simulink model "active_f2800137"  (R2024b)
settings: Solver=FixedStepDiscrete  StartTime=0.0  StopTime=inf  FixedStep=100e-6  RelTol=1e-3
model workspace (MAT data in the model file):
  ADC_FS = 4096
  ADC_VREF = 3.3
  G_CONST = 200
  IL_RATIO = 0.59
  IL_ZERO_V = 2.6365
  IPV_RATIO = 0.594
  IPV_ZERO_V = 2.6202
  ISENS_VPA = 0.1
  VOUT_RATIO = 0.021
  VPV_RATIO = 0.059
undefined symbols (not defined in the file or in its folder): Down, GPTRIP1SEL, GPTRIP2SEL, TZ1, TZ2, Up
libraries: c2802xlib x6, c2000lib x1, simulink x1
settings Model: ExtModeTrigDuration=8  Creator=YOGA Slim 7 Pro  LastModifiedBy=YOGA Slim 7 Pro
settings DataIOCC: SaveOutput=off  SignalLogging=off  DSMLogging=off  SaveTime=off  ReturnWorkspaceOutputs=off
settings OptimizationCC: DefaultParameterBehavior=Inlined  DefaultUnderspecifiedDataType=single  EnhancedBackFolding=on  PassReuseOutputArgsAs=Individual arguments  MaxStackSize=1024  OptimizeBlockOrder=speed  DifferentSizesBufferReuse=on  OptimizationCustomize=off  EfficientTunableParamExpr=on
settings DebuggingCC: ParameterTunabilityLossMsg=error
settings HardwareCC: ProdBitPerChar=16  ProdBitPerInt=16  ProdBitPerPointer=32  ProdBitPerSizeT=32  ProdBitPerPtrDiffT=32  ProdLargestAtomicInteger=Integer  ProdLargestAtomicFloat=None  ProdWordSize=16  ProdLongLongMode=on  ProdHWDeviceType=Texas Instruments->C2000
settings SFSimCC: MATLABDynamicMemAlloc=off
settings RTWCC: Description=Embedded Coder  SystemTargetFile=ert.tlc  HardwareBoard=TI F2800137 LaunchPad  TemplateMakefile=ert_default_tmf  Toolchain=Texas Instruments Code Composer Studio (C2000)  CodeProfilingSaveOptions=MetricsOnly
settings CodeAppCC: ForceParamTrailComments=on  IgnoreCustomStorageClasses=off  OperatorAnnotations=on  SimulinkDataObjDesc=on  SFDataObjDesc=on  InsertBlockDesc=on
settings ERTTargetCC: CodeReplacementLibrary=TI C28x  ExtModeTransport=4  ExtModeStaticAlloc=on  ExtModeAutomaticAllocSize=off  ExtModeStaticAllocSize=1000  ExtModeMexFile=ext_xcp  ExtModeIntrfLevel=Level2 - Open

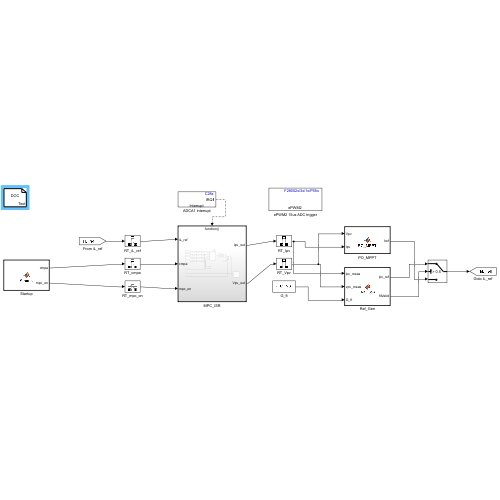
[thumbnail: Simulink's stored preview of the top-level diagram]
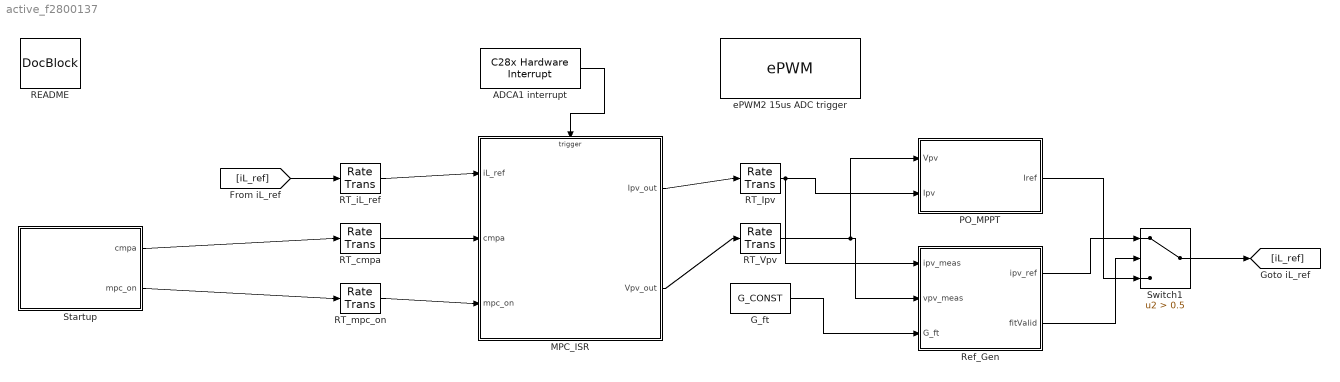
== system active_f2800137 ==
  ADCA1 interrupt : c2000lib/Scheduling/C28x Hardware Interrupt  irqnumbers=1  pienumbers=1  irqpriorities=30  irqpreempts=0  showinput=off  dspchiptype=C280X
  G_ft : Constant  Value=G_CONST  OutDataTypeStr=single  SampleTime=100e-6
  MPC_ISR : Subsystem  TreatAsAtomicUnit=on
  PO_MPPT : MATLAB Function  TreatAsAtomicUnit=on
  README : simulink/Model-Wide Utilities/DocBlock  DocumentType=Text
      content=|
      | active_f2800137 - controller of active.slx for the TMS320F2800137
      |
      | Gate output : ePWM1A = GPIO0
      | ADC-A inputs: iL=ADCIN2  Vin(Vpv)=ADCIN6  Vout=ADCIN3  Ipv=ADCIN5
      | Irradiance  : constant G_CONST = 200 W/m^2 (model workspace)
      | Scaling     : Model Explorer > Model Workspace
      |
      | MPC_Boost runs every 15 us in the ADCA1 interrupt (ePWM2 starts the
      | conversions). PO_MPPT and Ref_Gen run every 100 us. For t < 0.06 s
      | ePWM1A outputs the 30 kHz start-up PWM; afterwards the MPC switching
      | state S drives the pin directly.
  RT_Ipv : RateTransition  Deterministic=off  OutPortSampleTime=100e-6
  RT_Vpv : RateTransition  Deterministic=off  OutPortSampleTime=100e-6
  RT_cmpa : RateTransition  Deterministic=off  InitialCondition=200  OutPortSampleTimeOpt=Inherit
  RT_iL_ref : RateTransition  Deterministic=off  InitialCondition=4.9  OutPortSampleTimeOpt=Inherit
  RT_mpc_on : RateTransition  Deterministic=off  OutPortSampleTimeOpt=Inherit
  Ref_Gen : MATLAB Function  TreatAsAtomicUnit=on
  Startup : MATLAB Function  TreatAsAtomicUnit=on
  Switch1 : Switch  Criteria=u2 > Threshold  Threshold=0.5  SaturateOnIntegerOverflow=off  InputSameDT=off
  ePWM2 15us ADC trigger : c2802xlib/ePWM  PwmType=C2000_Type4_F28002x  useModule=ePWM2  ePWMxLINKTBPRD=Not Linked  periodUnits=Clock cycles  timerSource=Specify via dialog  timerPeriod_clk=1799  timerPeriod_sec=0.0001  tbshadow=Counter equals to zero  countingMode=Up  phaseActiveEnable=Disable  phaseDirection=Count down after sync  phaseActive=0  synchronizationEnable=off  dcaevt1Sync=off  dcbevt1Sync=off  synchronizationOption=Disable  dcbevt1SyncOut=off  dcaevt1SyncOut=off  cmpdSyncOut=off  cmpcSyncOut=off  cmpbSyncOut=off  zeroSyncOut=off  swfSyncOut=off  perSynchronizationOption=Counter equals to period (CTR=PRD)  clockPrescale=1  HSclockPrescale=1  enswap=off  ePWMxAStatus=off  ePWMxAactionLogic1=Set  ePWMxAactionLogic2=Clear  ePWMxAactionLogic3=Clear  ePWMxAactionLogic4=Set  ePWMxAactionLogic5=Do nothing  ePWMxAactionLogic6=Do nothing  ePWMxACSFenable=off  ePWMxACSFvalue=Forcing disable  ePWMxASFreload=Zero  ePWMxBStatus=off  ePWMxBactionLogic1=Set  ePWMxBactionLogic2=Clear  ePWMxBactionLogic3=Do nothing  ePWMxBactionLogic4=Do nothing  ePWMxBactionLogic5=Clear  ePWMxBactionLogic6=Set  ePWMxBCSFenable=off  ePWMxBCSFvalue=Forcing disable  ePWMxBSFreload=Zero  ePWNxBOutWay=off  ePWMxLINKCMPA=Not Linked  CMPAUnits=Clock cycles  CMPASource=Specify via dialog  CMPAValue_per=50  CMPAValue_clk=32000  enCMPAshadow=Counter equals to zero (CTR=Zero)  ePWMxLINKCMPB=Not Linked  CMPBUnits=Clock cycles  CMPBSource=Specify via dialog  CMPBValue_per=50  CMPBValue_clk=32000  enCMPBshadow=Counter equals to zero (CTR=Zero)  ePWMxLINKCMPC=Not Linked  CMPCUnits=Clock cycles  CMPCSource=Specify via dialog  CMPCValue_per=50  CMPCValue_clk=32000  enCMPCshadow=Counter equals to zero (CTR=Zero)  ePWMxLINKCMPD=Not Linked  CMPDUnits=Clock cycles  CMPDSource=Specify via dialog  CMPDValue_per=50  CMPDValue_clk=32000  enCMPDshadow=Counter equals to zero (CTR=Zero)  enableDBePWMxA=off  enableDBePWMxB=off  enhalfcycle=off  DBpolarity=Active high (AH)  DBedgeDelay=Positive  DBSource_ePWMxA=ePWMxA  DBSource_ePWMxB=ePWMxA  DBPeriodUnits=Clock cycles  DBperiodSource=Specify via dialog  REDperiod=0  FEDperiod=0  REDperiod_sec=0  FEDperiod_sec=0  LoadModeDBRED=Immediate without using shadow  LoadModeDBFED=Immediate without using shadow  adcstartModuleA=on  adcrequestEventA=First event  adcstartEventA=Counter equals to zero (CTR=Zero)  adcstartEventA_type2=Counter equals to zero (CTR=Zero)  adcstartModuleB=off  adcrequestEventB=First event  adcstartEventB=Counter equals to zero (CTR=Zero)  adcstartEventB_type2=Counter equals to zero (CTR=Zero)  intEn=off  intPrd=First event  intSel=Counter equals to zero (CTR=Zero)  intSel_type2=Counter equals to zero (CTR=Zero)  hrpe=off  enHRPWM=off  HRPWM_LoadMode=Counter equals to period (CTR=PRD)  HRPWM_CTLMode=Duty or Period control mode  HRPWM_EDGMode=Both edge  hrpeb=off  enHRPWMB=off  HRPWM_LoadModeB=Counter equals to zero (CTR=ZERO)  HRPWM_CTLModeB=Duty or Period control mode  HRPWM_EDGModeB=Both edge  enHRDBRED=off  enHRDBFED=off  enSFO=on  enautoconv=on  chopperEnable=off  chopperFrequency=1  chopperFirstwidth=1  chopperDuty=12.5%  tripZonesource=Specify via dialog  tzselOSHT1=off  tzselOSHT2=off  tzselOSHT3=off  tzselOSHT4=off  tzselOSHT5=off  tzselOSHT6=off  tzselOSHDCAEV1=off  tzselOSHDCBEV1=off  tzselCBC1=off  tzselCBC2=off  tzselCBC3=off  tzselCBC4=off  tzselCBC5=off  tzselCBC6=off  tzselCBCDCAEV2=off  tzselCBCDCBEV2=off  enTzOstIntr=off  enTzCbcIntr=off  enTzDCAEVT1Intr=off  enTzDCAEVT2Intr=off  enTzDCBEVT1Intr=off  enTzDCBEVT2Intr=off  tzclrCBCLatch=Counter equals to zero (CTR=Zero)  ePWMxAforced=No action  ePWMxBforced=No action  DCAEVT1forced=High  DCBEVT1forced=High  DCAEVT2forced=Low  DCBEVT2forced=Low  dcah=Trip Zone 1 input (TZ1)  dcal=Trip Zone 1 input (TZ1)  dcbh=Trip Zone 1 input (TZ1)  dcbl=Trip Zone 1 input (TZ1)  dcah_type2=GPTRIP1SEL/(TZ1)  dcal_type2=GPTRIP2SEL/(TZ2)  dcbh_type2=GPTRIP1SEL/(TZ1)  dcbl_type2=GPTRIP2SEL/(TZ2)  gendcaevt1=Event disabled  gendcaevt2=Event disabled  gendcbevt1=Event disabled  gendcbevt2=Event disabled  dcaevt1src=DCAEVT1 with sync  dcaevt2src=DCAEVT2 with sync  dcbevt1src=DCBEVT1 with sync  dcbevt2src=DCBEVT2 with sync  pulsesel=Counter equals to zero (CTR=Zero)  blankinv=off  blankoffset=0  blankwidth=0  evsrcsel=Filtered version of DCAEVT1 (DCAEVT1FILT)  encape=off
      settings: LibrarySourceBlock=c280013xlib/ePWM
  wires:
  ADCA1 interrupt/1 -> MPC_ISR/Trigger
  Startup/1(cmpa) -> RT_cmpa/1
  Startup/2(mpc_on) -> RT_mpc_on/1
  RT_iL_ref/1 -> MPC_ISR/1(iL_ref)
  RT_cmpa/1 -> MPC_ISR/2(cmpa)
  RT_mpc_on/1 -> MPC_ISR/3(mpc_on)
  MPC_ISR/1(Ipv_out) -> RT_Ipv/1
  MPC_ISR/2(Vpv_out) -> RT_Vpv/1
  RT_Vpv/1 -> PO_MPPT/1(Vpv), Ref_Gen/2(vpv_meas)
  RT_Ipv/1 -> PO_MPPT/2(Ipv), Ref_Gen/1(ipv_meas)
  G_ft/1 -> Ref_Gen/3(G_ft)
  Ref_Gen/1(ipv_ref) -> Switch1/1
  Ref_Gen/2(fitValid) -> Switch1/2
  PO_MPPT/1(Iref) -> Switch1/3
  Switch1/1 -> [iL_ref]
  [iL_ref] -> RT_iL_ref/1

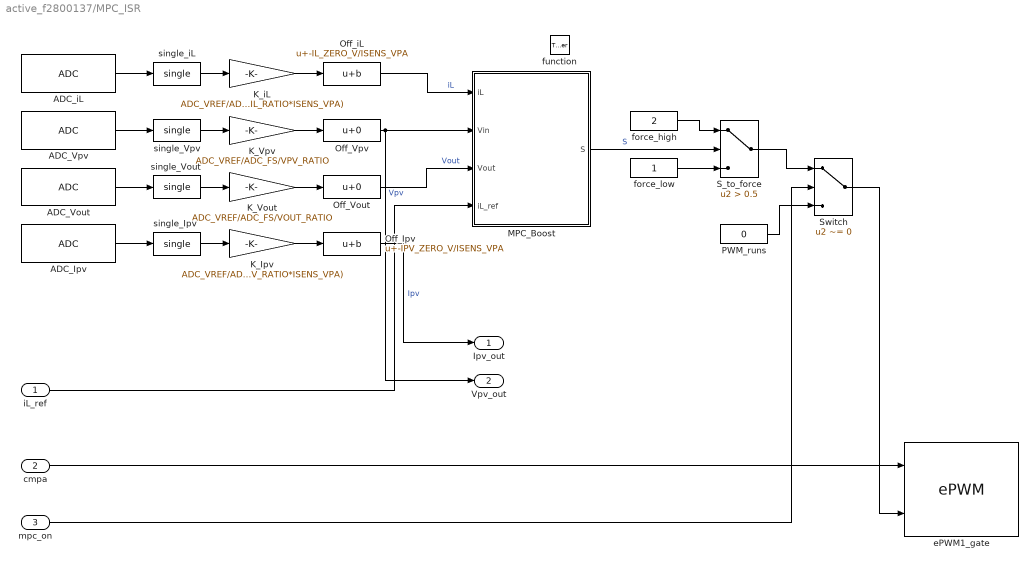
== system active_f2800137/MPC_ISR ==
  iL_ref : Inport
  cmpa : Inport  Port=2
  mpc_on : Inport  Port=3
  function : TriggerPort  TriggerType=function-call  VariantControl=(inherit)  PortDimensions=1
  ADC_Ipv : c2802xlib/ADC  blkParamProc=C2000_Type5_001x  ADCModule=A  samplingMode=Single sample mode  ADCResolution=12-bit (Single-ended input)  useSOC1=SOC3  useSOC2=SOC0_SOC1  SOCAcquisitionWindow=40  SOCTriggerSource=ePWM2_ADCSOCA  SOCInterruptTrigger=No ADCINT  Ts=-1  dType=uint16  postInterrupt=on  interruptSel=ADCINT1  ADCINTContinuous=on  endma=off  chdma=1  conv1=ADCINA0  conv2=ADCINA0 and ADCINB0  conv1_Type4=ADCIN5  conv2_Type4=ADCIN0 and ADCIN1
      settings: LibrarySourceBlock=c280013xlib/ADC
  ADC_Vout : c2802xlib/ADC  blkParamProc=C2000_Type5_001x  ADCModule=A  samplingMode=Single sample mode  ADCResolution=12-bit (Single-ended input)  useSOC1=SOC2  useSOC2=SOC0_SOC1  SOCAcquisitionWindow=40  SOCTriggerSource=ePWM2_ADCSOCA  SOCInterruptTrigger=No ADCINT  Ts=-1  dType=uint16  postInterrupt=off  interruptSel=ADCINT1  ADCINTContinuous=on  endma=off  chdma=1  conv1=ADCINA0  conv2=ADCINA0 and ADCINB0  conv1_Type4=ADCIN3  conv2_Type4=ADCIN0 and ADCIN1
      settings: LibrarySourceBlock=c280013xlib/ADC
  ADC_Vpv : c2802xlib/ADC  blkParamProc=C2000_Type5_001x  ADCModule=A  samplingMode=Single sample mode  ADCResolution=12-bit (Single-ended input)  useSOC1=SOC1  useSOC2=SOC0_SOC1  SOCAcquisitionWindow=40  SOCTriggerSource=ePWM2_ADCSOCA  SOCInterruptTrigger=No ADCINT  Ts=-1  dType=uint16  postInterrupt=off  interruptSel=ADCINT1  ADCINTContinuous=on  endma=off  chdma=1  conv1=ADCINA0  conv2=ADCINA0 and ADCINB0  conv1_Type4=ADCIN6  conv2_Type4=ADCIN0 and ADCIN1
      settings: LibrarySourceBlock=c280013xlib/ADC
  ADC_iL : c2802xlib/ADC  blkParamProc=C2000_Type5_001x  ADCModule=A  samplingMode=Single sample mode  ADCResolution=12-bit (Single-ended input)  useSOC1=SOC0  useSOC2=SOC0_SOC1  SOCAcquisitionWindow=40  SOCTriggerSource=ePWM2_ADCSOCA  SOCInterruptTrigger=No ADCINT  Ts=-1  dType=uint16  postInterrupt=off  interruptSel=ADCINT1  ADCINTContinuous=on  endma=off  chdma=1  conv1=ADCINA0  conv2=ADCINA0 and ADCINB0  conv1_Type4=ADCIN2  conv2_Type4=ADCIN0 and ADCIN1
      settings: LibrarySourceBlock=c280013xlib/ADC
  K_Ipv : Gain  Gain=ADC_VREF/ADC_FS/(IPV_RATIO*ISENS_VPA)  ParamDataTypeStr=single  OutDataTypeStr=single
  K_Vout : Gain  Gain=ADC_VREF/ADC_FS/VOUT_RATIO  ParamDataTypeStr=single  OutDataTypeStr=single
  K_Vpv : Gain  Gain=ADC_VREF/ADC_FS/VPV_RATIO  ParamDataTypeStr=single  OutDataTypeStr=single
  K_iL : Gain  Gain=ADC_VREF/ADC_FS/(IL_RATIO*ISENS_VPA)  ParamDataTypeStr=single  OutDataTypeStr=single
  MPC_Boost : MATLAB Function  TreatAsAtomicUnit=on
  Off_Ipv : Bias  Bias=-IPV_ZERO_V/ISENS_VPA  SaturateOnIntegerOverflow=off
  Off_Vout : Bias  SaturateOnIntegerOverflow=off
  Off_Vpv : Bias  SaturateOnIntegerOverflow=off
  Off_iL : Bias  Bias=-IL_ZERO_V/ISENS_VPA  SaturateOnIntegerOverflow=off
  PWM_runs : Constant  Value=0  OutDataTypeStr=uint16
  S_to_force : Switch  Criteria=u2 > Threshold  Threshold=0.5  SaturateOnIntegerOverflow=off  InputSameDT=off
  Switch : Switch  Criteria=u2 ~= 0  SaturateOnIntegerOverflow=off  InputSameDT=off
  ePWM1_gate : c2802xlib/ePWM  PwmType=C2000_Type4_F28002x  useModule=ePWM1  ePWMxLINKTBPRD=Not Linked  periodUnits=Clock cycles  timerSource=Specify via dialog  timerPeriod_clk=2000  timerPeriod_sec=0.0001  tbshadow=Counter equals to zero  countingMode=Up-Down  phaseActiveEnable=Disable  phaseDirection=Count down after sync  phaseActive=0  synchronizationEnable=off  dcaevt1Sync=off  dcbevt1Sync=off  synchronizationOption=Disable  dcbevt1SyncOut=off  dcaevt1SyncOut=off  cmpdSyncOut=off  cmpcSyncOut=off  cmpbSyncOut=off  zeroSyncOut=off  swfSyncOut=off  perSynchronizationOption=Counter equals to period (CTR=PRD)  clockPrescale=1  HSclockPrescale=1  enswap=off  ePWMxAStatus=on  ePWMxAactionLogic1=Set  ePWMxAactionLogic2=Clear  ePWMxAactionLogic3=Clear  ePWMxAactionLogic4=Set  ePWMxAactionLogic5=Do nothing  ePWMxAactionLogic6=Do nothing  ePWMxACSFenable=on  ePWMxACSFvalue=Forcing disable  ePWMxASFreload=Immediate  ePWMxBStatus=off  ePWMxBactionLogic1=Set  ePWMxBactionLogic2=Clear  ePWMxBactionLogic3=Do nothing  ePWMxBactionLogic4=Do nothing  ePWMxBactionLogic5=Clear  ePWMxBactionLogic6=Set  ePWMxBCSFenable=off  ePWMxBCSFvalue=Forcing disable  ePWMxBSFreload=Immediate  ePWNxBOutWay=off  ePWMxLINKCMPA=Not Linked  CMPAUnits=Clock cycles  CMPASource=Input port  CMPAValue_per=50  CMPAValue_clk=200  enCMPAshadow=Counter equals to zero (CTR=Zero)  ePWMxLINKCMPB=Not Linked  CMPBUnits=Clock cycles  CMPBSource=Specify via dialog  CMPBValue_per=50  CMPBValue_clk=32000  enCMPBshadow=Counter equals to zero (CTR=Zero)  ePWMxLINKCMPC=Not Linked  CMPCUnits=Clock cycles  CMPCSource=Specify via dialog  CMPCValue_per=50  CMPCValue_clk=32000  enCMPCshadow=Counter equals to zero (CTR=Zero)  ePWMxLINKCMPD=Not Linked  CMPDUnits=Clock cycles  CMPDSource=Specify via dialog  CMPDValue_per=50  CMPDValue_clk=32000  enCMPDshadow=Counter equals to zero (CTR=Zero)  enableDBePWMxA=off  enableDBePWMxB=off  enhalfcycle=off  DBpolarity=Active high (AH)  DBedgeDelay=Positive  DBSource_ePWMxA=ePWMxA  DBSource_ePWMxB=ePWMxA  DBPeriodUnits=Clock cycles  DBperiodSource=Specify via dialog  REDperiod=0  FEDperiod=0  REDperiod_sec=0  FEDperiod_sec=0  LoadModeDBRED=Immediate without using shadow  LoadModeDBFED=Immediate without using shadow  adcstartModuleA=off  adcrequestEventA=First event  adcstartEventA=Counter equals to zero (CTR=Zero)  adcstartEventA_type2=Counter equals to zero (CTR=Zero)  adcstartModuleB=off  adcrequestEventB=First event  adcstartEventB=Counter equals to zero (CTR=Zero)  adcstartEventB_type2=Counter equals to zero (CTR=Zero)  intEn=off  intPrd=First event  intSel=Counter equals to zero (CTR=Zero)  intSel_type2=Counter equals to zero (CTR=Zero)  hrpe=off  enHRPWM=off  HRPWM_LoadMode=Counter equals to period (CTR=PRD)  HRPWM_CTLMode=Duty or Period control mode  HRPWM_EDGMode=Both edge  hrpeb=off  enHRPWMB=off  HRPWM_LoadModeB=Counter equals to zero (CTR=ZERO)  HRPWM_CTLModeB=Duty or Period control mode  HRPWM_EDGModeB=Both edge  enHRDBRED=off  enHRDBFED=off  enSFO=on  enautoconv=on  chopperEnable=off  chopperFrequency=1  chopperFirstwidth=1  chopperDuty=12.5%  tripZonesource=Specify via dialog  tzselOSHT1=off  tzselOSHT2=off  tzselOSHT3=off  tzselOSHT4=off  tzselOSHT5=off  tzselOSHT6=off  tzselOSHDCAEV1=off  tzselOSHDCBEV1=off  tzselCBC1=off  tzselCBC2=off  tzselCBC3=off  tzselCBC4=off  tzselCBC5=off  tzselCBC6=off  tzselCBCDCAEV2=off  tzselCBCDCBEV2=off  enTzOstIntr=off  enTzCbcIntr=off  enTzDCAEVT1Intr=off  enTzDCAEVT2Intr=off  enTzDCBEVT1Intr=off  enTzDCBEVT2Intr=off  tzclrCBCLatch=Counter equals to zero (CTR=Zero)  ePWMxAforced=No action  ePWMxBforced=No action  DCAEVT1forced=High  DCBEVT1forced=High  DCAEVT2forced=Low  DCBEVT2forced=Low  dcah=Trip Zone 1 input (TZ1)  dcal=Trip Zone 1 input (TZ1)  dcbh=Trip Zone 1 input (TZ1)  dcbl=Trip Zone 1 input (TZ1)  dcah_type2=GPTRIP1SEL/(TZ1)  dcal_type2=GPTRIP2SEL/(TZ2)  dcbh_type2=GPTRIP1SEL/(TZ1)  dcbl_type2=GPTRIP2SEL/(TZ2)  gendcaevt1=Event disabled  gendcaevt2=Event disabled  gendcbevt1=Event disabled  gendcbevt2=Event disabled  dcaevt1src=DCAEVT1 with sync  dcaevt2src=DCAEVT2 with sync  dcbevt1src=DCBEVT1 with sync  dcbevt2src=DCBEVT2 with sync  pulsesel=Counter equals to zero (CTR=Zero)  blankinv=off  blankoffset=0  blankwidth=0  evsrcsel=Filtered version of DCAEVT1 (DCAEVT1FILT)  encape=off
      settings: LibrarySourceBlock=c280013xlib/ePWM
  force_high : Constant  Value=2  OutDataTypeStr=uint16
  force_low : Constant  OutDataTypeStr=uint16
  single_Ipv : DataTypeConversion  OutDataTypeStr=single  SaturateOnIntegerOverflow=off  RndMeth=Floor
  single_Vout : DataTypeConversion  OutDataTypeStr=single  SaturateOnIntegerOverflow=off  RndMeth=Floor
  single_Vpv : DataTypeConversion  OutDataTypeStr=single  SaturateOnIntegerOverflow=off  RndMeth=Floor
  single_iL : DataTypeConversion  OutDataTypeStr=single  SaturateOnIntegerOverflow=off  RndMeth=Floor
  Ipv_out : Outport
  Vpv_out : Outport  Port=2
  wires:
  ADC_iL/1 -> single_iL/1
  single_iL/1 -> K_iL/1
  K_iL/1 -> Off_iL/1
  ADC_Vpv/1 -> single_Vpv/1
  single_Vpv/1 -> K_Vpv/1
  K_Vpv/1 -> Off_Vpv/1
  ADC_Vout/1 -> single_Vout/1
  single_Vout/1 -> K_Vout/1
  K_Vout/1 -> Off_Vout/1
  ADC_Ipv/1 -> single_Ipv/1
  single_Ipv/1 -> K_Ipv/1
  K_Ipv/1 -> Off_Ipv/1
  Off_iL/1 -> MPC_Boost/1(iL)  "iL"
  Off_Vpv/1 -> Vpv_out/1, MPC_Boost/2(Vin)  "Vpv"
  Off_Vout/1 -> MPC_Boost/3(Vout)  "Vout"
  iL_ref/1 -> MPC_Boost/4(iL_ref)
  force_high/1 -> S_to_force/1
  MPC_Boost/1(S) -> S_to_force/2  "S"
  force_low/1 -> S_to_force/3
  S_to_force/1 -> Switch/1
  mpc_on/1 -> Switch/2
  PWM_runs/1 -> Switch/3
  cmpa/1 -> ePWM1_gate/1
  Switch/1 -> ePWM1_gate/2
  Off_Ipv/1 -> Ipv_out/1  "Ipv"

== matlab function active_f2800137/Startup ==
  settings: updateMethod=DISCRETE  sampleTime=100e-6
  data: cmpa output; mpc_on output
function [cmpa, mpc_on] = Startup()
% Start-up sequence of active.slx, called every 100 us.
%   Ramp (0.1 + 31.2*t) -> Saturation [0.1, 0.722] : duty of the 30 kHz PWM
%   Step at 0.06 s                                : hands the gate to the MPC
%   cmpa   : ePWM1 compare value (TBPRD = 2000 counts = duty 1)
%   mpc_on : true for t >= 0.06 s

Ts     = single(100e-6);     % call period (s)
Nstep  = uint16(600);        % 0.06 s / 100 us
TBPRD  = single(2000);       % ePWM1 period register, 30 kHz up-down

persistent k
if isempty(k)
    k = uint16(0);
end

t = single(k) * Ts;
D = min(max(single(0.1) + single(31.2) * t, single(0.1)), single(0.722));

cmpa   = uint16(D * TBPRD);
mpc_on = k >= Nstep;

if k < Nstep
    k = k + uint16(1);
end

end

== matlab function active_f2800137/MPC_ISR/MPC_Boost ==
  data: iL input; S output; Vin input; Vout input; iL_ref input
function S = MPC_Boost(iL, Vin, Vout, iL_ref)
% Finite-control-set MPC for the boost converter (one-step prediction).
% Single precision: all four inputs must be single.

Ts = single(15e-6);          % controller period (s)
L  = single(0.00166914);     % boost inductance (H)
RL = single(0);              % inductor resistance (ohm)
wf = single(0.001);          % switching penalty

States = single([1; 0]);

persistent S_old
if isempty(S_old)
    S_old = single(0);
end

g_op = single(inf);
n_op = uint16(1);

for n = uint16(1):uint16(2)
    iL_k1 = iL + (Ts/L) * (Vin - iL*RL - Vout*(single(1) - States(n)));
    g = (iL_ref - iL_k1)^2 + wf*(States(n) - S_old)^2;
    if g < g_op
        g_op = g;
        n_op = n;
    end
end

S = States(n_op);
S_old = S;

end

== matlab function active_f2800137/PO_MPPT ==
  data: Vpv input; Iref output; Ipv input
function Iref = PO_MPPT(Vpv, Ipv)
% Perturb-and-observe MPPT producing an inductor-current reference.
% Single precision: both inputs must be single.

persistent Pprev Vprev Irefprev n

Imin     = single(0.10);     % A
Imax     = single(5);        % A
Irefinit = single(4.9);      % A, reference held during startup
deltaI   = single(0.02);     % A, perturbation step
Ijump    = single(0.5);      % A, re-synchronisation threshold
Nstart   = uint16(600);      % last call index of the startup hold

P = Vpv * Ipv;

if isempty(n)
    Pprev = P;
    Vprev = Vpv;
    Irefprev = Irefinit;
    n = uint16(0);
end

if n <= Nstart
    % Startup: hold the initial reference
    Iref = Irefinit;
    n = n + uint16(1);
elseif abs(Ipv - Irefprev) > Ijump
    % Reference is far from the measured current: re-synchronise
    Iref = min(max(Ipv, Imin), Imax);
else
    % P&O step
    if (P - Pprev > 0) == (Vpv - Vprev > 0)
        Iref = Irefprev - deltaI;
    else
        Iref = Irefprev + deltaI;
    end
    Iref = min(max(Iref, Imin), Imax);
end

Pprev = P;
Vprev = Vpv;
Irefprev = Iref;

end

== matlab function active_f2800137/Ref_Gen ==
  data: ipv_meas input; ipv_ref output; vpv_meas input; G_ft input; fitValid output
function [ipv_ref, fitValid] = Ref_Gen(ipv_meas, vpv_meas, G_ft)
% Irradiance-normalised curve-fit MPPT using the future irradiance G_ft.
% Single precision: all three inputs must be single.
%   ipv_ref  : PV / inductor current reference (A)
%   fitValid : 1 when ipv_ref comes from a validated fitted model

% ------------------------- Constants ------------------------------
G_REF   = single(1000.0);   % W/m^2, normalisation irradiance
Isc_STC = single(5.1);      % A
Voc_STC = single(31.0);     % V
G_MIN   = single(20.0);     % W/m^2, below this the forecast is invalid

A_G    = single(1.35);      % V, logarithmic irradiance voltage coefficient
Rs_eff = single(0.50);      % ohm, effective series-resistance correction

Ts_MPPT = 100e-6;           % function-call period (s)
T_COLLECT_START = 0.10;     % s, ignore samples before this time
collectStartCalls = uint32(max(1, round(T_COLLECT_START/Ts_MPPT)));

MAX_HISTORY = 7;
MIN_HISTORY = uint32(5);
historySeparation = single(0.015);  % A, minimum distance of a new stored point
minPairGap = single(0.010);         % A
minSpan    = single(0.040);         % A
minGramDet = single(1e-8);

SETTLE_WINDOW_CALLS = 10;
stableWindowIRange  = single(0.20); % A
stableWindowVRange  = single(0.75); % V

voltageEnvelopeTol = single(0.75);  % V
maxFitRmsError = single(1.00);      % V
maxFitAbsError = single(2.00);      % V
supportTolNorm = single(0.04);      % A

GjumpFrac = single(0.10);
FIT_CONFIRM_CALLS    = uint32(5);
FIT_FAIL_GRACE_CALLS = uint32(5);
DeltaI     = single(0.020);         % A, candidate spacing
alphaDP    = single(0.20);          % low-pass coefficient for P(I+) - P(I-)
P_deadband = single(0.05);          % W
GRID_N     = uint32(101);           % grid points of the initial MPP search

ZERO = single(0);
ONE  = single(1);

ipv_ref  = ZERO;
fitValid = ZERO;

% ------------------------- Persistent state -----------------------
persistent InormBuf VnormBuf nHist
persistent Gprev GprevValid callCount initialized
persistent recentI recentV recentCount recentIndex
persistent modelValid cLast ImeanLast IscaleLast
persistent IminLast ImaxLast VminLast VmaxLast
persistent lastRefNorm lastRefNormValid DeltaP_filt
persistent fitGoodCount fitBadCount fitReady

forecastValid = ~isnan(G_ft) && ~isinf(G_ft) && G_ft >= G_MIN;

if isempty(initialized) || ~forecastValid
    InormBuf = zeros(1, MAX_HISTORY, 'single');
    VnormBuf = zeros(1, MAX_HISTORY, 'single');
    nHist = uint32(0);
    Gprev = ZERO;
    GprevValid = false;
    callCount = uint32(0);
    recentI = zeros(1, SETTLE_WINDOW_CALLS, 'single');
    recentV = zeros(1, SETTLE_WINDOW_CALLS, 'single');
    recentCount = uint32(0);
    recentIndex = uint32(0);
    modelValid = false;
    cLast = zeros(3, 1, 'single');
    ImeanLast = ZERO;
    IscaleLast = ONE;
    IminLast = ZERO;
    ImaxLast = ZERO;
    VminLast = ZERO;
    VmaxLast = ZERO;
    lastRefNorm = ZERO;
    lastRefNormValid = false;
    DeltaP_filt = ZERO;
    fitGoodCount = uint32(0);
    fitBadCount = uint32(0);
    fitReady = false;
    initialized = true;
end

if ~forecastValid
    return;
end

% Counts calls only until the collection start is reached (no overflow).
if callCount < collectStartCalls
    callCount = callCount + uint32(1);
end

% ------------------------- Reference limits -----------------------
Isc_target = Isc_STC * G_ft / G_REF;
Iref_min = max(single(0.02) * Isc_target, single(0.001));
Iref_max = max(single(0.97) * Isc_target, Iref_min + single(1e-4));
Iref_max = min(Iref_max, single(0.999) * Isc_STC);
Iref_max = max(Iref_max, Iref_min + single(1e-4));
Iref_max = min(Iref_max, Isc_STC);

% ------------------------- Irradiance step detection --------------
stepDetected = false;
if GprevValid && Gprev >= G_MIN
    stepDetected = abs(G_ft - Gprev) >= GjumpFrac * max(Gprev, G_MIN);
end

measurementValid = ~isnan(ipv_meas) && ~isinf(ipv_meas) && ipv_meas > ZERO && ...
                   ~isnan(vpv_meas) && ~isinf(vpv_meas) && vpv_meas > ZERO;

% ------------------------- Settling window ------------------------
measurementSettled = false;
if stepDetected
    DeltaP_filt = ZERO;
    recentI = zeros(1, SETTLE_WINDOW_CALLS, 'single');
    recentV = zeros(1, SETTLE_WINDOW_CALLS, 'single');
    recentCount = uint32(0);
    recentIndex = uint32(0);
end

if measurementValid
    recentIndex = recentIndex + uint32(1);
    if recentIndex > SETTLE_WINDOW_CALLS
        recentIndex = uint32(1);
    end
    recentI(recentIndex) = ipv_meas;
    recentV(recentIndex) = vpv_meas;
    if recentCount < SETTLE_WINDOW_CALLS
        recentCount = recentCount + uint32(1);
    end

    if recentCount >= SETTLE_WINDOW_CALLS
        measurementSettled = ...
            (max(recentI) - min(recentI)) <= stableWindowIRange && ...
            (max(recentV) - min(recentV)) <= stableWindowVRange;
    end
end

% ------------------------- Normalise and store sample -------------
% The PV sample of this call belongs to the previous forecast Gprev.
if measurementValid && callCount >= collectStartCalls && ...
        measurementSettled && GprevValid && Gprev >= G_MIN

    normRatio = G_REF / Gprev;
    newInorm = ipv_meas * normRatio;
    newVnorm = vpv_meas + A_G * log(normRatio) ...
               - Rs_eff * (newInorm - ipv_meas);

    sampleValid = ~isnan(newInorm) && ~isinf(newInorm) && ...
        ~isnan(newVnorm) && ~isinf(newVnorm) && newInorm > ZERO && ...
        newVnorm > ZERO && newVnorm <= single(1.5) * Voc_STC;

    if sampleValid
        if nHist == 0
            nHist = uint32(1);
            InormBuf(1) = newInorm;
            VnormBuf(1) = newVnorm;
        else
            novelSample = true;
            closestIndex = uint32(1);
            closestDistance = single(inf);
            for k = uint32(1):nHist
                dist = abs(newInorm - InormBuf(k));
                if dist < closestDistance
                    closestDistance = dist;
                    closestIndex = k;
                end
                if dist < historySeparation
                    novelSample = false;
                end
            end

            if novelSample
                if nHist < MAX_HISTORY
                    nHist = nHist + uint32(1);
                    InormBuf(nHist) = newInorm;
                    VnormBuf(nHist) = newVnorm;
                else
                    InormBuf(closestIndex) = newInorm;
                    VnormBuf(closestIndex) = newVnorm;
                end
            end
        end
    end
end

% ------------------------- Fit normalised V-I curve ---------------
% V = c(1)*x^2 + c(2)*x + c(3), x = (I - Imean)/Iscale
fitSucceeded = false;
fitImean = ZERO;
fitIscale = ONE;
cFit = zeros(3, 1, 'single');
fitImin = ZERO;
fitImax = ZERO;
fitVmin = ZERO;
fitVmax = ZERO;

if measurementValid && nHist >= MIN_HISTORY
    nHistF = single(nHist);

    fitImin = InormBuf(1);
    fitImax = InormBuf(1);
    fitVmin = VnormBuf(1);
    fitVmax = VnormBuf(1);
    minGap = single(inf);
    for i = uint32(1):nHist
        fitImin = min(fitImin, InormBuf(i));
        fitImax = max(fitImax, InormBuf(i));
        fitVmin = min(fitVmin, VnormBuf(i));
        fitVmax = max(fitVmax, VnormBuf(i));
        for j = i+uint32(1):nHist
            minGap = min(minGap, abs(InormBuf(i) - InormBuf(j)));
        end
    end

    if ~(minGap < minPairGap || (fitImax - fitImin) < minSpan)
        fitImean = ZERO;
        for i = uint32(1):nHist
            fitImean = fitImean + InormBuf(i);
        end
        fitImean = fitImean / nHistF;

        fitIscale = ZERO;
        for i = uint32(1):nHist
            fitIscale = max(fitIscale, abs(InormBuf(i) - fitImean));
        end

        if ~(fitIscale <= single(1e-6))
            s1 = ZERO; s2 = ZERO; s3 = ZERO; s4 = ZERO;
            t0 = ZERO; t1 = ZERO; t2 = ZERO;
            for i = uint32(1):nHist
                xi = (InormBuf(i) - fitImean) / fitIscale;
                vi = VnormBuf(i);
                x2 = xi * xi;
                s1 = s1 + xi;
                s2 = s2 + x2;
                s3 = s3 + x2 * xi;
                s4 = s4 + x2 * x2;
                t0 = t0 + vi;
                t1 = t1 + xi * vi;
                t2 = t2 + x2 * vi;
            end

            M = [s4, s3, s2; s3, s2, s1; s2, s1, nHistF];
            rhs = [t2; t1; t0];
            detM = det(M);

            if ~(isnan(detM) || isinf(detM) || abs(detM) < minGramDet)
                cTry = M \ rhs;
                if all(~isnan(cTry)) && all(~isinf(cTry))
                    sumErr2 = ZERO;
                    maxAbsErr = ZERO;
                    for i = uint32(1):nHist
                        xi = (InormBuf(i) - fitImean) / fitIscale;
                        err = cTry(1)*xi*xi + cTry(2)*xi + cTry(3) - VnormBuf(i);
                        sumErr2 = sumErr2 + err*err;
                        maxAbsErr = max(maxAbsErr, abs(err));
                    end
                    rmsErr = sqrt(sumErr2 / nHistF);
                    if ~(rmsErr > maxFitRmsError || maxAbsErr > maxFitAbsError)
                        cFit = cTry;
                        fitSucceeded = true;
                    end
                end
            end
        end
    end
end

% ------------------------- Keep the last validated model ----------
if fitSucceeded
    cLast = cFit;
    ImeanLast = fitImean;
    IscaleLast = fitIscale;
    IminLast = fitImin;
    ImaxLast = fitImax;
    VminLast = fitVmin;
    VmaxLast = fitVmax;
    modelValid = true;

    if fitGoodCount < FIT_CONFIRM_CALLS
        fitGoodCount = fitGoodCount + uint32(1);
    end
    fitBadCount = uint32(0);
    if fitGoodCount >= FIT_CONFIRM_CALLS
        fitReady = true;
    end
else
    fitGoodCount = uint32(0);
    if fitReady
        fitBadCount = fitBadCount + uint32(1);
        if fitBadCount >= FIT_FAIL_GRACE_CALLS
            fitReady = false;
            fitBadCount = uint32(0);
        end
    else
        fitBadCount = uint32(0);
    end
end

% ------------------------- Translate to G_ft and choose I+/I- -----
futureReferenceValid = false;
if modelValid
    rFuture = G_ft / G_REF;
    logR = log(rFuture);

    % First valid model: grid search for the MPP of the translated curve,
    % restricted to the measured current support.
    if ~lastRefNormValid
        supportLow = max(Iref_min, rFuture * IminLast);
        supportHigh = min(Iref_max, rFuture * ImaxLast);
        bestP = single(-inf);
        bestI = ZERO;
        bestGridIndex = uint32(0);

        if supportHigh > supportLow
            for gi = uint32(0):(GRID_N - uint32(1))
                frac = single(gi) / single(GRID_N - uint32(1));
                Itry = supportLow + frac * (supportHigh - supportLow);
                Ibase = Itry / rFuture;
                xtry = (Ibase - ImeanLast) / IscaleLast;
                Vbase = cLast(1)*xtry*xtry + cLast(2)*xtry + cLast(3);
                Vtry = Vbase + A_G*logR - Rs_eff*(Itry - Ibase);
                if Ibase >= IminLast && Ibase <= ImaxLast && ...
                        Vbase >= VminLast - voltageEnvelopeTol && ...
                        Vbase <= VmaxLast + voltageEnvelopeTol && ...
                        Vtry > ZERO && Vtry <= single(1.2)*Voc_STC
                    Ptry = Itry * Vtry;
                    if ~isnan(Ptry) && ~isinf(Ptry) && Ptry > bestP
                        bestP = Ptry;
                        bestI = Itry;
                        bestGridIndex = gi;
                    end
                end
            end
        end

        if bestGridIndex <= 1 || bestGridIndex >= (GRID_N - uint32(1)) || bestP <= ZERO
            modelValid = false;
            fitReady = false;
            fitGoodCount = uint32(0);
        else
            lastRefNorm = bestI / rFuture;
            lastRefNormValid = true;
            DeltaP_filt = ZERO;
        end
    end

    if modelValid && lastRefNormValid
        targetSpan = rFuture * (ImaxLast - IminLast);
        DeltaILocal = min(DeltaI, single(0.45) * targetSpan);
        centerLow = max(Iref_min, rFuture*IminLast + DeltaILocal);
        centerHigh = min(Iref_max, rFuture*ImaxLast - DeltaILocal);

        if ~(centerHigh <= centerLow || DeltaILocal <= single(1e-6))
            center = lastRefNorm * rFuture;
            center = min(max(center, centerLow), centerHigh);
            Iplus = min(max(center + DeltaILocal, Iref_min), Iref_max);
            Iminus = min(max(center - DeltaILocal, Iref_min), Iref_max);

            IplusBase = Iplus / rFuture;
            IminusBase = Iminus / rFuture;
            xPlus = (IplusBase - ImeanLast) / IscaleLast;
            xMinus = (IminusBase - ImeanLast) / IscaleLast;
            VplusBase = cLast(1)*xPlus*xPlus + cLast(2)*xPlus + cLast(3);
            VminusBase = cLast(1)*xMinus*xMinus + cLast(2)*xMinus + cLast(3);
            Vplus = VplusBase + A_G*logR - Rs_eff*(Iplus - IplusBase);
            Vminus = VminusBase + A_G*logR - Rs_eff*(Iminus - IminusBase);

            plusSupported = IplusBase >= IminLast-supportTolNorm && ...
                IplusBase <= ImaxLast+supportTolNorm && ...
                VplusBase >= VminLast-voltageEnvelopeTol && ...
                VplusBase <= VmaxLast+voltageEnvelopeTol && ...
                Vplus > ZERO && Vplus <= single(1.2)*Voc_STC;
            minusSupported = IminusBase >= IminLast-supportTolNorm && ...
                IminusBase <= ImaxLast+supportTolNorm && ...
                VminusBase >= VminLast-voltageEnvelopeTol && ...
                VminusBase <= VmaxLast+voltageEnvelopeTol && ...
                Vminus > ZERO && Vminus <= single(1.2)*Voc_STC;

            if plusSupported
                Pplus = Iplus * Vplus;
            else
                Pplus = single(-1);
            end
            if minusSupported
                Pminus = Iminus * Vminus;
            else
                Pminus = single(-1);
            end

            if Pplus > ZERO && Pminus > ZERO && ...
                    ~isnan(Pplus) && ~isinf(Pplus) && ...
                    ~isnan(Pminus) && ~isinf(Pminus)
                DeltaP = Pplus - Pminus;
                if stepDetected
                    DeltaP_filt = DeltaP;
                else
                    DeltaP_filt = (ONE - alphaDP)*DeltaP_filt + alphaDP*DeltaP;
                end

                if DeltaP_filt > P_deadband
                    ipv_ref = Iplus;
                elseif DeltaP_filt < -P_deadband
                    ipv_ref = Iminus;
                else
                    ipv_ref = center;
                end

                lastRefNorm = ipv_ref / rFuture;
                futureReferenceValid = true;
            else
                ipv_ref = center;
            end
        end
    end
end

% ------------------------- Fallback reference ---------------------
if ~modelValid || ~lastRefNormValid
    if lastRefNormValid
        ipv_ref = min(max(lastRefNorm * (G_ft/G_REF), Iref_min), Iref_max);
    else
        ipv_ref = min(max(single(0.80)*Isc_target, Iref_min), Iref_max);
    end
end

if fitReady && modelValid && lastRefNormValid && futureReferenceValid
    fitValid = ONE;
end

Gprev = G_ft;
GprevValid = true;

end
